simulink model "HexaMotor_Force_FF"  (R2022b)
settings: Solver=FixedStepAuto  StartTime=0.0  StopTime=120  RelTol=1e-3  EnableMultiTasking=on
model workspace (MAT data in the model file):
  sampleRate = 0.005
libraries: arduinolib x3, arduinomotorcarrierlib x2, eeGeneralControl x2, slpidlib x1, simulink x1
settings Model: ExtModeTrigDuration=2  Creator=bkhusain  LastModifiedBy=arkad
settings SolverCC: AlgebraicLoopSolver=TrustRegion
settings DataIOCC: ReturnWorkspaceOutputs=off
settings OptimizationCC: EnhancedBackFolding=on  PassReuseOutputArgsThreshold=0  MaxStackSize=64  OptimizeBlockOrder=speed  DifferentSizesBufferReuse=on  OptimizationCustomize=off
settings DebuggingCC: ParameterOverflowMsg=none  ParameterUnderflowMsg=error  ParameterPrecisionLossMsg=none  ParameterTunabilityLossMsg=error  UnconnectedInputMsg=warning  UnconnectedOutputMsg=warning  UnconnectedLineMsg=warning  SFMachineParentedDataDiag=warning
settings HardwareCC: ProdBitPerPointer=32  ProdBitPerSizeT=32  ProdBitPerPtrDiffT=32  ProdLargestAtomicInteger=Long  ProdLargestAtomicFloat=Double  ProdWordSize=32  ProdHWDeviceType=ARM Compatible->ARM Cortex
settings ModelReferenceCC: EnableRefExpFcnMdlSchedulingChecks=on
settings SFSimCC: MATLABDynamicMemAlloc=off
settings RTWCC: Description=Embedded Coder  SystemTargetFile=ert.tlc  HardwareBoard=Arduino MKRZero  TLCOptions=-aInlineSetEventsForThisBaseRateFcn=TLC_FALSE -aSuppressMultiTaskScheduler=TLC_FALSE -aRateBasedStepFcn=1  TemplateMakefile=ert_default_tmf  Toolchain=Arduino ARM  BuildConfiguration=Faster Runs  DLArmComputeVersion=19.05
settings CodeAppCC: ForceParamTrailComments=on  OperatorAnnotations=on
settings ERTTargetCC: ERTCustomFileBanners=off  SupportContinuousTime=on  SupportNonInlinedSFcns=on  RemoveResetFunc=off  SupportVariableSizeSignals=on  ModelStepFunctionPrototypeControlCompliant=off  ExtModeTransport=3  ExtModeStaticAlloc=on  ExtModeAutomaticAllocSize=off  ExtModeStaticAllocSize=8192  ExtModeMexFile=ext_xcp  ExtModeIntrfLevel=Level2 - Open

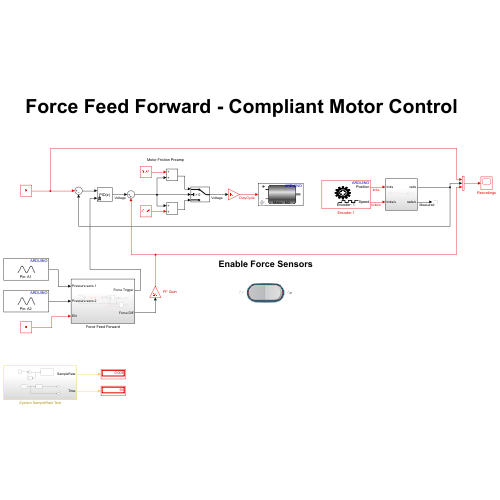
[thumbnail: Simulink's stored preview of the top-level diagram]
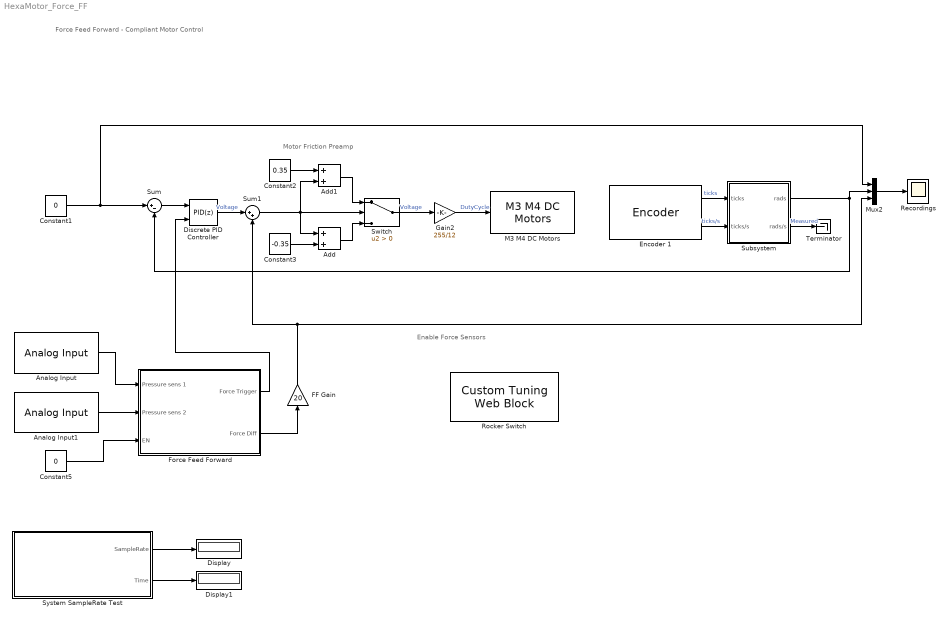
== system HexaMotor_Force_FF ==
  note: Enable Force Sensors
  note: Motor Friction Preamp
  note: Force Feed Forward - Compliant Motor Control
  Add : Sum
  Add1 : Sum
  Analog Input : arduinolib/Analog Input  pinNumber=1  ReadResultsOnly=off  ConversionTriggerSource=Software  ExternalTriggerType=uint32( 0 )  OutputDataType=uint16  EnableConversionCompleteNotify=off  EnableOuputStatus=off  SampleTime=sampleRate  blockPlatform=arduino
  Analog Input1 : arduinolib/Analog Input  pinNumber=2  ReadResultsOnly=off  ConversionTriggerSource=Software  ExternalTriggerType=uint32( 0 )  OutputDataType=uint16  EnableConversionCompleteNotify=off  EnableOuputStatus=off  SampleTime=sampleRate  blockPlatform=arduino
  Constant1 : Constant  Value=0  SampleTime=sampleRate
  Constant2 : Constant  Value=0.35  SampleTime=sampleRate
  Constant3 : Constant  Value=-0.35  SampleTime=sampleRate
  Constant5 : Constant  Value=0  SampleTime=sampleRate
  Discrete PID Controller : slpidlib/PID Controller  Controller=PID  Form=Parallel  TimeDomain=Discrete-time  UseExternalTs=off  SampleTime=sampleRate  IntegratorMethod=Forward Euler  FilterMethod=Forward Euler  ControllerParametersSource=internal  P=10  I=1  UseKiTs=off  D=0.1  N=100  UseFilter=on  TunerSelectOption=Transfer Function Based (PID Tuner App)  InitialConditionSource=internal  InitialConditionForIntegrator=0  InitialConditionForFilter=0  DifferentiatorICPrevScaledInput=0  ExternalReset=level  TrackingMode=off  Kt=1  LimitOutput=off  SatLimitsSource=internal  UpperSaturationLimit=inf  LowerSaturationLimit=-inf  LinearizeAsGain=off  AntiWindupMode=none  Kb=1  LimitIntegrator=off  UpperIntegratorSaturationLimit=inf  LowerIntegratorSaturationLimit=-inf  POutMin=[]  POutMax=[]  IOutMin=[]  IOutMax=[]  DOutMin=[]  DOutMax=[]  NOutMin=[]  NOutMax=[]  SumOutMin=[]  SumOutMax=[]  SaturationOutMin=[]  SaturationOutMax=[]  PParamMin=[]  PParamMax=[]  IParamMin=[]  IParamMax=[]  DParamMin=[]  DParamMax=[]  NParamMin=[]  NParamMax=[]  KbParamMin=[]  KbParamMax=[]  KtParamMin=[]  KtParamMax=[]  KbOutMin=[]  KbOutMax=[]  KtOutMin=[]  KtOutMax=[]  IntegratorOutMin=[]  IntegratorOutMax=[]  FilterOutMin=[]  FilterOutMax=[]  SumI1OutMin=[]  SumI1OutMax=[]  SumI2OutMin=[]  SumI2OutMax=[]  SumI3OutMin=[]  SumI3OutMax=[]  SumI4OutMin=[]  SumI4OutMax=[]  SumDOutMin=[]  SumDOutMax=[]  DifferentiatorOutMin=[]  DifferentiatorOutMax=[]  FilterDiffOutCoefMin=[]  FilterDiffOutCoefMax=[]  ReciprocalOutMin=[]  ReciprocalOutMax=[]  SumDenOutMin=[]  SumDenOutMax=[]  SumNumOutMin=[]  SumNumOutMax=[]  DivideOutMin=[]  DivideOutMax=[]  UdiffTsProdOutMin=[]  UdiffTsProdOutMax=[]  NTsProdOutMin=[]  NTsProdOutMax=[]  UintegralTsProdOutMin=[]  UintegralTsProdOutMax=[]  UngainTsProdOutMin=[]  UngainTsProdOutMax=[]  ClampingZeroOutDataTypeStr=Inherit: Inherit via back propagation  ClampingZeroOutMin=[]  ClampingZeroOutMax=[]  FilterDenConstantOutDataTypeStr=Inherit: Inherit via back propagation  FilterDenConstantOutMin=[]  FilterDenConstantOutMax=[]  PCopyOutDataTypeStr=Inherit: Inherit via back propagation  PCopyOutMin=[]  PCopyOutMax=[]  NCopyOutDataTypeStr=Inherit: Inherit via back propagation  NCopyOutMin=[]  NCopyOutMax=[]  IntegratorContinuousStateAttributes=''  IntegratorStateMustResolveToSignalObject=off  IntegratorRTWStateStorageClass=Auto  FilterContinuousStateAttributes=''  FilterStateMustResolveToSignalObject=off  FilterRTWStateStorageClass=Auto  ParallelPVariant=InternalParameters  IdealPVariant=Disabled  IVariant=InternalParameters  DVariant=InternalParameters  IntegratorVariant=Discrete  SatVariant=Disabled  AWVariant=Passthrough  PCopyVariant=Disabled  TRVariant=Disabled  FdbkBlocksVariant=Forward  IdealPFdbkVariant=Disabled  SatFdbkVariant=Disabled  DerivativeFilterVariant=ForwardEulerFilter  NVariant=InternalParameters  NCopyVariant=Disabled  FilterICVariant=InternalICsFilter  IntegratorICVariant=InternalICs  ExternalResetVariant=ExternalReset  TRSumVariant=Passthrough  SumFdbkVariant=Disabled  SumVariant=Sum_PID  TsampFilterVariant=InternalTs  TsampNgainVariant=Passthrough  TsampIntegralVariant=Passthrough  ExternalSaturationOutDataTypeStr=Inherit: Same as second input
      settings: LibrarySourceBlock=simulink/Discrete/Discrete PID Controller
  Display : Display
  Display1 : Display
  Encoder 1 : arduinomotorcarrierlib/Encoder  SlaveAddress=uint8( hex2dec( '66' ) )  blockPlatform=ARDUINO  Encoder=1  ShowSpeed=on  ResetOption=on  SampleTime=sampleRate
  FF Gain : Gain  Gain=20
  Force Feed Forward : Subsystem
  Gain2 : Gain  Gain=255/12
  M3 M4 DC Motors : arduinomotorcarrierlib/M3 M4 DC Motors  MotorNumber=M3  forwardPinNumber=3  reversePinNumber=2
  Mux2 : Mux  Inputs=3
  Recordings : Scope
  Rocker Switch : CustomTuningWebBlock  LabelPosition=Hide  ShowInitialText=on  Configuration="{\"type\":\"Switch\",\"settings\":{\"BindingType\":\"param\",\"backgroundColor\":[0,0,255,\"1\"],\"backgroundOffset\":0.14,\"fixedAspectRatio\":\"on\",\"foregroundColor\":[234,234,234],\"showBackgroundColor\":false,\"variant\":\"rocker\"},\"components\":[{\"name\":\"CustomSwitchStateComponent\",\"settings\":{\"position\":[0,0,1,1],\"states\":[{\"HitRegion\":{\"position\":[0,0,0.5,1]},\"Image\":{\"position\":[0.13,0,1,0.75],\"size\":[1,0.75],\"src\":\"data:image/svg+xml;base64,PHN2ZyB4bWxucz0iaHR0cDovL3d3dy53My5vcmcvMjAwMC9zdmciIHhtbG5zOnhsaW5rPSJodHRwOi8vd3d3LnczLm9yZy8xOTk5L3hsaW5rIiB2aWV3Qm94PSIwIDAgNzUgMjQuOCI+PGRlZnM+PHN0eWxlPi5jbHMtMXtmaWxsOnVybCgjcmFkaWFsLWdyYWRpZW50KTt9LmNscy0ye2ZpbGw6dXJsKCNyYWRpYWwtZ3JhZGllbnQtMik7fS5jbHMtM3tzdHJva2U6I2IyMDAwMDtzdHJva2Utd2lkdGg6MC4yNXB4O2ZpbGw6dXJsKCNsaW5lYXItZ3JhZGllbnQpO30uY2xzLTR7ZmlsbDp1cmwoI2xpbmVhci1ncmFkaWVudC0yKTt9LmNs ...(+3576 chars)\",\"srcOrientation\":\"Right\"},\"Label\":{\"color\":[0.5019607843137255,0.5019607843137255,0.5019607843137255],\"icon\":{\"size\":[0,0],\"src\":[],\"srcOrientation\":\"Right\"},\"iconPlacement\":\"left\",\"opacity\":1,\"position\":[0.5,0.08],\"show\":true,\"text\":{\"content\":\"Off\",\"font\":\"Helvetica\",\"fontSize\":14}},\"Value\":0},{\"HitRegion\":{\"position\":[0,0.5,0.5,1]},\"Image\":{\"position\":[0.13,0,1,0.75],\"size\":[1,0.75],\"src\":\"data:image/svg+xml;base64,PHN2ZyB4bWxucz0iaHR0cDovL3d3dy53My5vcmcvMjAwMC9zdmciIHhtbG5zOnhsaW5rPSJodHRwOi8vd3d3LnczLm9yZy8xOTk5L3hsaW5rIiB2aWV3Qm94PSIwIDAgNzUgMjQuOCI+PGRlZnM+PHN0eWxlPi5jbHMtMXtmaWxsOnVybCgjcmFkaWFsLWdyYWRpZW50KTt9LmNscy0ye2ZpbGw6dXJsKCNyYWRpYWwtZ3JhZGllbnQtMik7fS5jbHMtM3tzdHJva2U6I2IyMDAwMDtzdHJva2Utd2lkdGg6MC4yNXB4O2ZpbGw6dXJsKCNsaW5lYXItZ3JhZGllbnQpO30uY2xzLTR7ZmlsbDp1cmwoI2xpbmVhci1ncmFkaWVudC0yKTt9LmNs ...(+3520 chars)\",\"srcOrientation\":\"Right\"},\"Label\":{\"color\":[0.5019607843137255,0.5019607843137255,0.5019607843137255],\"icon\":{\"size\":[0,0],\"src\":[],\"srcOrientation\":\"Right\"},\"iconPlacement\":\"left\",\"opacity\":1,\"position\":[0.5,0.92],\"show\":true,\"text\":{\"content\":\"On\",\"font\":\"Helvetica\",\"fontSize\":14}},\"Value\":1}]}},{\"name\":\"BackgroundImageComponent\",\"settings\":{\"image\":{\"size\":[155,70],\"src\":\"default\",\"srcOrientation\":\"Right\"},\"position\":[0,0,1,1],\"scaleMode\":\"0\"}},{\"name\":\"ForegroundImageComponent\",\"settings\":{\"image\":{\"size\":[0,0],\"src\":\"default\",\"srcOrientation\":[]},\"isForeground\":1,\"position\":[0,0,1,1],\"scaleMode\":\"0\"}}]}"
  Subsystem : Subsystem
  Sum : Sum  Inputs=|+-
  Sum1 : Sum  Inputs=|++
  Switch : Switch  Criteria=u2 > Threshold  SaturateOnIntegerOverflow=off  InputSameDT=off
  System SampleRate Test : Subsystem
  Terminator : Terminator
  wires:
  Gain2/1 -> M3 M4 DC Motors/1  "DutyCycle"
  System SampleRate Test/1(SampleRate) -> Display/1
  System SampleRate Test/2(Time) -> Display1/1
  Encoder 1/1 -> Subsystem/1(ticks)  "ticks"
  Encoder 1/2 -> Subsystem/2(ticks/s)  "ticks/s"
  Sum/1 -> Discrete PID Controller/1
  Add1/1 -> Switch/1
  Constant3/1 -> Add/2
  Add/1 -> Switch/3
  Constant2/1 -> Add1/1
  Switch/1 -> Gain2/1  "Voltage"
  Mux2/1 -> Recordings/1
  Subsystem/2(rads/s) -> Terminator/1  "Measured"
  Subsystem/1(rads) -> Mux2/2, Sum/2
  Constant1/1 -> Sum/1, Mux2/1
  Discrete PID Controller/1 -> Sum1/1  "Voltage"
  Sum1/1 -> Switch/2, Add1/2, Add/1
  Analog Input/1 -> Force Feed Forward/1(Pressure sens 1)
  Analog Input1/1 -> Force Feed Forward/2(Pressure sens 2)
  Force Feed Forward/2(Force Diff) -> FF Gain/1
  FF Gain/1 -> Mux2/3, Sum1/2
  Force Feed Forward/1(Force Trigger) -> Discrete PID Controller/2
  Constant5/1 -> Force Feed Forward/3(EN)

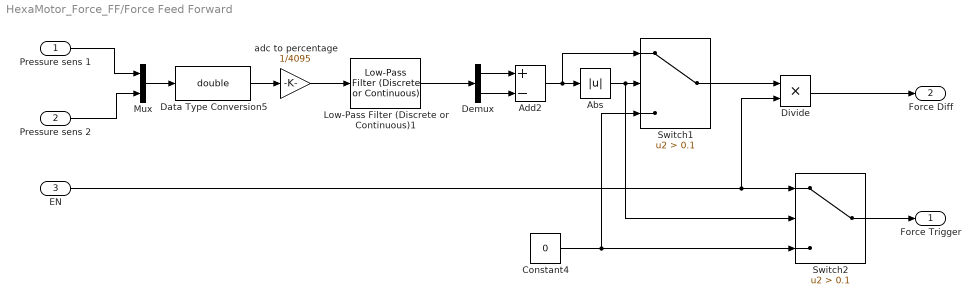
== system HexaMotor_Force_FF/Force Feed Forward ==
  Pressure sens 1 : Inport
  Pressure sens 2 : Inport  Port=2
  EN : Inport  Port=3
  Abs : Abs  SaturateOnIntegerOverflow=off
  Add2 : Sum  Inputs=+-
  Constant4 : Constant  Value=0  SampleTime=sampleRate
  Data Type Conversion5 : DataTypeConversion  OutDataTypeStr=double  SaturateOnIntegerOverflow=off  RndMeth=Floor
  Demux : Demux  Outputs=2
  Divide : Product  Inputs=**
  Low-Pass Filter (Discrete or Continuous)1 : eeGeneralControl/Low-Pass Filter (Discrete or Continuous)  K=1  T=0.1  B=inf  A=-inf  init_option=Inherited from block input  x0=0  Ts=sampleRate
  Mux : Mux  Inputs=2
  Switch1 : Switch  Criteria=u2 > Threshold  Threshold=0.1  SaturateOnIntegerOverflow=off  InputSameDT=off
  Switch2 : Switch  Criteria=u2 > Threshold  Threshold=0.1  SaturateOnIntegerOverflow=off  InputSameDT=off
  adc to percentage : Gain  Gain=1/4095
  Force Trigger : Outport
  Force Diff : Outport  Port=2
  wires:
  Add2/1 -> Switch1/1, Abs/1
  Low-Pass Filter (Discrete or Continuous)1/1 -> Demux/1
  Abs/1 -> Switch2/2, Switch1/2
  Data Type Conversion5/1 -> adc to percentage/1
  adc to percentage/1 -> Low-Pass Filter (Discrete or Continuous)1/1
  Demux/1 -> Add2/1
  Demux/2 -> Add2/2
  Mux/1 -> Data Type Conversion5/1
  Pressure sens 2/1 -> Mux/2
  Pressure sens 1/1 -> Mux/1
  EN/1 -> Switch2/1, Divide/2
  Constant4/1 -> Switch1/3, Switch2/3
  Switch2/1 -> Force Trigger/1
  Switch1/1 -> Divide/1
  Divide/1 -> Force Diff/1

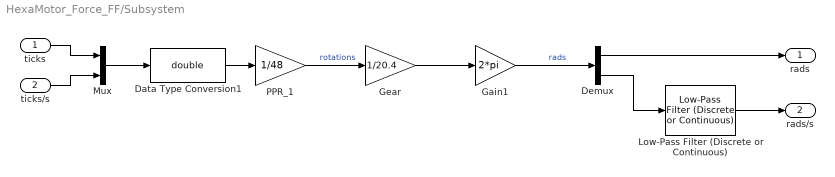
== system HexaMotor_Force_FF/Subsystem ==
  ticks : Inport
  ticks/s : Inport  Port=2
  Data Type Conversion1 : DataTypeConversion  OutDataTypeStr=double  SaturateOnIntegerOverflow=off  RndMeth=Floor
  Demux : Demux  Outputs=2
  Gain1 : Gain  Gain=2*pi
  Gear : Gain  Gain=1/20.4
  Low-Pass Filter (Discrete or Continuous) : eeGeneralControl/Low-Pass Filter (Discrete or Continuous)  K=1  T=0.05  B=inf  A=-inf  init_option=Inherited from block input  x0=0  Ts=sampleRate
  Mux : Mux  Inputs=2
  PPR_1 : Gain  Gain=1/48
  rads : Outport
  rads/s : Outport  Port=2
  wires:
  PPR_1/1 -> Gear/1  "rotations"
  Data Type Conversion1/1 -> PPR_1/1
  Mux/1 -> Data Type Conversion1/1
  ticks/1 -> Mux/1
  Gear/1 -> Gain1/1
  ticks/s/1 -> Mux/2
  Gain1/1 -> Demux/1  "rads"
  Demux/1 -> rads/1
  Demux/2 -> Low-Pass Filter (Discrete or Continuous)/1
  Low-Pass Filter (Discrete or Continuous)/1 -> rads/s/1

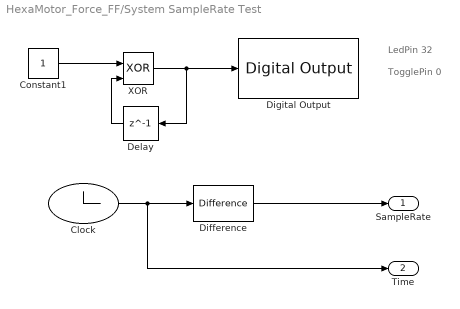
== system HexaMotor_Force_FF/System SampleRate Test ==
  note: LedPin 32
  note: TogglePin 0
  Clock : Clock
      settings: Decimation=3
  Constant1 : Constant  SampleTime=sampleRate
  Delay : Delay  DelayLength=1  InitialCondition=0  SampleTime=sampleRate
  Difference : simulink/Quick Insert/Discrete/Difference  ICPrevInput=0.0  OutMin=[]  OutMax=[]  OutDataType=fixdt(1, 16)  OutScaling=2^-10  DoSatur=off
  Digital Output : arduinolib/Digital Output  pinNumber=0  Direction=output  blockPlatform=arduino
  XOR : Logic  Operator=XOR  IconShape=distinctive  AllPortsSameDT=off  OutDataTypeStr=boolean
  SampleRate : Outport
  Time : Outport  Port=2
  wires:
  XOR/1 -> Delay/1, Digital Output/1
  Constant1/1 -> XOR/1
  Delay/1 -> XOR/2
  Clock/1 -> Time/1, Difference/1
  Difference/1 -> SampleRate/1
